simulink model "EV6_LUT_FourWheel_EV6Battery77p4kWh_PowerCorrected"  (R2024a)
settings: Solver=ode4  StartTime=0  StopTime=60  FixedStep=0.001  RelTol=1e-3
PreLoadFcn:
  | VSS_BICYCLE=Simulink.Variant('Dual=0');
  | VSS_DUAL=Simulink.Variant('Dual=1');
  | Dual=1;
  | load('DriveCycle2.mat')
PostLoadFcn:
  | if any(exist('dsrtsu_mdlpostloadfcn', 'file') ~= 0), dsrtsu_mdlpostloadfcn('Execute', bdroot); end
InitFcn:
  | , if any(exist('rtifpga_mdlclblib', 'file') ~= 0), rtifpga_mdlclblib('Init', bdroot); end,
  | , if any(exist('dsmpb_private', 'file') ~= 0), dsmpb_private('dsmpb_mdlclblib', 'Init', bdroot); end,
  | load('DriveCycle2.mat')
model workspace (MAT data in the model file):
  DiffRatio = 10.65
  EV6_2023_BattBranchCapacity_Ah = 55.5236728838
  EV6_2023_BattEnergy_kWh = 77.4
  EV6_2023_BattNominalVoltage_V = 697
  EV6_2023_BattNumCellsParallel = 2
  EV6_2023_BattNumCellsSeries = 192
  EV6_2023_BattOpenVoltCapBpts = [0 0.1 0.2 0.3 0.4 0.5 0.6 0.7 0.8 0.9 1]
  EV6_2023_BattOpenVoltTbl = [2.96762142548 3.40364281191 3.47417488548 3.54470541822 3.61523441014 3.68576186124 3.75628777151 3.82681214095 3.94527005036 4.07101207308 4.2120755254]
  EV6_2023_BattPackCapacity_Ah = 111.047345768
  EV6_2023_BattResistSocBpts = [0 0.2 0.4 0.6 0.8 1]
  EV6_2023_BattResistTbl = [0.0163620057716 0.0118174152018 0.00807187352333 0.00375663957972 0.00266904525531 0.00103635901355 0.0019014404175 0.0172368903217 0.0121226074867 0.00758541551769 0.00474065349228 0.00337561163613 ... (42 elements, 7x6)]
  EV6_2023_BattResistTempBpts = [243.1 253.1 263.1 273.1 283.1 298.1 313.1]
  EV6_2023_InitialPackOCV_V = 726.471714233
  EV6_2023_InitialSOC = 0.638878863672
  EV6_BattCellCapacity_Ah = 60.3
  EV6_BattInitialSOC = 0.638878863672
  EV6_BattOCV_Cell_V = [2.96762142548 3.40364281191 3.47417488548 3.54470541822 3.61523441014 3.68576186124 3.75628777151 3.82681214095 3.94527005036 4.07101207308 4.2120755254]
  EV6_BattOCV_SOC = [0 0.1 0.2 0.3 0.4 0.5 0.6 0.7 0.8 0.9 1]
  EV6_BattPackCapacity_Ah = 120.6
  EV6_BattParallelCells = 2
  EV6_BattResistanceSOC = [0 0.2 0.4 0.6 0.8 1]
  EV6_BattResistanceTable_Ohm = [0.0163620057716 0.0118174152018 0.00807187352333 0.00375663957972 0.00266904525531 0.00103635901355 0.0019014404175 0.0172368903217 0.0121226074867 0.00758541551769 0.00474065349228 0.00337561163613 ... (42 elements, 7x6)]
  EV6_BattResistanceTemp_K = [243.1 253.1 263.1 273.1 283.1 298.1 313.1]
  EV6_BattSeriesCells = 192
  EV6_FinalDriveRatio = 10.65
  EV6_TargetPackResistance_Ohm = 0.132763804608
  Gas = 0.383333333333
undefined symbols (not defined in the file): accel_bp_mps2, AccelCmd, ActTqLF_Nm_, ActTqLR_Nm_, ActTqRF_Nm_, ActTqRR_Nm_, BattChargeLimitMaxPwr, BattChargeLimitSocBpts, BattChargeLimitTbl, BattDischargeLimitSocBpts, BattDischargeLimitTbl, BattDischargeMaxPwr, BrakeMaxPrs, BrakeMaxTrq, ChassisDistCg2FrontAxle, ChassisDistCg2RearAxle, ChassisVehMass, CltchCmd, CoastDown, DecelCmd, DiscIntNeverNeededParam, EnvGravCnst, EnvPrs, EnvTemp, EV6_RegenTorqueGain, EV6_TractionTorqueGain, front_share_regen_3d, front_share_traction_3d, FuelSpecificGrav, GearCmd, h, InitStates, lgSw, limitedMCT, MCT, MtrEffSpdBpts, MtrEffTbl, MtrEffTrqBpts, MtrPwrMax, MtrTrqMax, out_1, pMCT, RealSimPara, Ref_speed, Ref_time, regen_torque_bp_Nm, speed_bp_kph, SteeringCmd, SupvsryCtrlRegenBrkCutOffTbl, SupvsryCtrlRegenSpdBpts, TestScnrioCycleNum, traction_torque_bp_Nm, US06, VEH
libraries: VSIGenLib x65, simulink x54, etargetslib x38, dsmpblib x24, vehdynlibtire x12, autolibshared x11, vehdynlibsuspension x7, vehdynlibtirecommon x7, autolibpowerinfoutils x6, autolibutils x5, autolibsharedcoupling x4, autolibmappedmotor x4
(part 5 of 19)

== system EV6_LUT_FourWheel_EV6Battery77p4kWh_PowerCorrected/Vehicle Under Test1/Vehicle/Motor_R ==
  SupvsryCtrl : Inport
  MtrSpd : Inport  Port=2
  Bus Creator1 : BusCreator  Inputs=1
  Bus Creator2 : BusCreator  Inputs=4
  Bus Selector1 : BusSelector  OutputSignals=Volt
  Bus Selector2 : BusSelector  OutputSignals=MtrTrqCmd
  Bus Selector3 : BusSelector  OutputSignals=PwrInfo.PwrTrnsfrd.PwrMtr,PwrInfo.PwrTrnsfrd.PwrBus
  Mach-E Motor : autolibmappedmotor/Mapped Motor  port_config=Speed  param_by=Maximum torque and power  w_t=[ 0 375 750 800 ]  T_t=[0.09 0.08 0.07 0]  torque_max=800  power_max=358000  Tc=0.01  param_loss=Tabulated efficiency data  eff=100  w_eff=375  T_eff=0.08  Piron=0  Pbase=0  w_eff_bp=MtrEffSpdBpts.*pi/30  T_eff_bp=MtrEffTrqBpts  Temp_eff_bp=[233.15 293.15 373.15]  losses_table=[1 2;3 4]  losses_table_3d=cat(3,[1.49 1.67 2.21 3.10; 0.42 0.69 1.14 2.03; 0.06 0.24 0.78 1.68; 0.42 0.69 1.14 2.03; 1.49 1.67 2.21 3.10],[1.49 1.67 2.21 3.10; 0.42 0.69 1.14 2.03; 0.06 0.24 0.78 1.68; 0.42 0.69 1.14 2.03; 1.49 1.67 2.21 3.10],[1.49 1.67 2.21 3.10; 0.42 0.69 1.14 2.03; 0.06 0.24 0.78 1.68; 0.42 0.69 1.14 2.03; 1.49 1.67 2.21 3.10])  efficiency_table=MtrEffTbl*0.94  efficiency_table_3d=cat(3,[95 95 95 95; 95 95 95 95; 95 95 95 95; 95 95 95 95; 95 95 95 95],[95 95 95 95; 95 95 95 95; 95 95 95 95; 95 95 95 95; 95 95 95 95],[95 95 95 95; 95 95 95 95; 95 95 95 95; 95 95 95 95; 95 95 95 95])  J=5e-6  b=1e-5  omega_o=0  T_t_extended=[0 0.07 0.08 0.09 0.08 0.07 0]  w_t_extended=[-800 -750 -375 0 375 750 800]  KLossIron=0  KLossCopper=0  x_w_eff_vec=[-1047.1975511966 -942.477796076938 -837.758040957278 -733.038285837618 -628.318530717959 -523.598775598299 -418.879020478639 -314.159265358979 -285.714285713875 -209.43951023932 -104.71975511966 0 104.71975511966 209.43951023932 285.714285713875 314.159265358979 418.879020478639 523.598775598299 628.318530717959 733.038285837618 837.758040957278 942.477796076938 1047.1975511966]  x_T_eff_vec=[-360 -334.285714285714 -308.571428571429 -282.857142857143 -257.142857142857 -231.428571428571 -205.714285714286 -180 -154.285714285714 -128.571428571429 -102.857142857143 -77.1428571428572 -51.4285714285714 -25.7142857142857 0 25.7142857142857 51.4285714285714 77.1428571428572 102.857142857143 128.571428571429 154.285714285714 180 205.714285714286 231.428571428571 257.142857142857 282.857142857143 308.571428571429 334.285714285714 360]  x_tmp_eff_vec=[-0.09 -0.06 -0.03 0 0.03 0.06 0.09]  x_losses_mat=[54250.1517943165 50375.1409518653 46500.1301094142 42625.119266963 38750.1084245118 34875.0975820605 31000.0867396095 27125.0758971582 23250.065054707 19375.054212256 15500.0433698047 12629.4764797412 9803.55154311708 6774.11181875432 0 5412.5153431847 8293.80460547705 10921.9712596802 13550.1379138833 16937.6723923542 20325.2068708249 23712.7413492957 27100.2758277666 30487.8103062373 33875.3447847082 37262.879263179 40650.4137416499 44037.9482201206 47425.4826985915;44696.230836134 41503.6429192672 38311.0550024006 35118.4670855338 31925.8791686671 28733.2912518003 25540.7033349337 22348.115418067 19155.5275012002 15962.9395843336 12770.3516674669 9577.76375060014 6975.01951641212 6096.70063687888 0 4871.26380886623 6097.56206124747 8462.91205003029 11283.8827333737 14104.8534167172 16925.8241000605 19746.794783404 22567.7654667475 25388.7361500908 28209.7068334343 31030.6775167777 33851.6482001212 36672.6188834645 39493.589566808;36137.1105685043 33555.8883850397 30974.6662015752 28393.4440181105 25812.2218346459 23230.9996511813 20649.7774677168 18068.5552842522 15487.3331007875 12906.110917323 10324.8887338584 8513.56777831124 6200.01734792188 5419.28945500345 0 4330.01227454776 5420.05516555331 7522.58848891581 9220.12563933554 11525.1570491694 13830.1884590033 16135.2198688372 18440.2512786711 20745.2826885049 23050.3140983388 25355.3455081727 27660.3769180066 29965.4083278404 32270.4397376744;31619.9717474413 29361.4023369097 27102.8329263783 24844.2635158467 22585.6941053152 20327.1246947836 18068.5552842522 15809.9858737206 13551.4164631891 11292.8470526576 9034.27764212609 7449.37180602233 5425.01517943165 4741.87827312802 0 3788.76074022929 4742.54826985915 6582.26492780134 8067.6099344186 10084.5124180233 12101.4149016279 14118.3173852325 16135.2198688372 18152.1223524418 20169.0248360465 22185.9273196511 24202.8298032558 26219.7322868604 28236.6347704651;27102.8329263782 25166.9162887798 23230.9996511814 21295.0830135829 19359.1663759844 17423.249738386 15487.3331007876 13551.4164631891 11615.4998255906 9679.58318799226 8513.56777831124 6385.17583373343 4650.01301094141 4064.46709125259 0 3247.50920591082 4065.04137416498 5641.94136668686 7522.58848891582 8643.86778687709 10372.6413442524 12101.4149016279 13830.1884590033 15558.9620163787 17287.7355737541 19016.5091311295 20745.282688505 22474.0562458803 24202.8298032558;22585.6941053152 20972.4302406498 19359.1663759845 17745.9025113191 16132.6386466537 14519.3747819883 12906.110917323 11292.8470526576 9679.58318799221 8066.31932332688 7094.63981525937 5320.97986144452 3875.01084245118 3387.05590937716 0 2706.25767159235 3387.53447847082 4701.61780557238 6268.82374076318 7203.22315573091 8643.86778687704 10084.5124180232 11525.1570491694 12965.8016803156 14406.4463114618 15847.0909426079 17287.7355737541 18728.3802049003 20169.0248360465;19864.9914827262 18446.0635196743 17027.1355566225 15608.2075935706 14189.2796305187 12770.3516674668 11351.423704415 9932.4957413631 8513.56777831121 7094.63981525938 5675.71185220749 4256.78388915562 3100.00867396094 2709.64472750173 0 2165.00613727388 2710.02758277665 3761.29424445791 5015.05899261055 6268.82374076319 7522.58848891579 8776.35323706844 10030.1179852211 11283.8827333737 12537.6474815263 13791.412229679 15045.1769778316 16298.9417259842 17552.7064741369;20587.4582405459 19116.9255090783 17646.3927776108 16175.8600461432 12629.4764797412 11366.528831767 10103.581183793 8137.52276914747 6975.01951641211 5812.51626367679 4650.01301094142 3788.84294392236 2525.89529594824 2032.23354562629 0 1623.75460295541 2184.39425193603 3276.59137790406 4065.04137416499 5081.30171770625 6097.56206124746 7113.82240478872 8737.57700774416 9829.77413371214 10921.9712596802 13684.7775990372 14928.8482898587 16172.9189806802 17416.9896715018;18723.4042552922 17386.0182370571 16048.6322188219 14711.2462005868 11485.9634880614 10337.3671392553 9188.77079044916 8040.174441643 6891.57809283685 5742.98174403074 4594.38539522458 ...(+6536 chars)]  x_losses_mat_3d=[37.8947368421052 25.2631578947368 12.6315789473684 0 12 24 36;18.9473684210526 12.6315789473684 6.3157894736842 0 5.99999999999999 12 18;0 0 0 0 0 0 0;18 12 5.99999999999999 0 6.3157894736842 12.6315789473684 18.9473684210526;36 24 12 0 12.6315789473684 25.2631578947368 37.8947368421052]  CalLossMapData={}  CalLossWithTempMapData={}  aMode=aMode  RefBlkName='autolibmappedmotor/Mapped Motor'
  Mapped Motor : autolibmappedmotor/Mapped Motor  port_config=Speed  param_by=Maximum torque and power  w_t=[ 0 375 750 800 ]  T_t=[0.09 0.08 0.07 0]  torque_max=MtrTrqMax  power_max=MtrPwrMax  Tc=MtrTrqTimeCnst  param_loss=Tabulated efficiency data  eff=100  w_eff=375  T_eff=0.08  Piron=0  Pbase=0  w_eff_bp=MtrEffSpdBpts.*pi/30  T_eff_bp=MtrEffTrqBpts  Temp_eff_bp=[233.15 293.15 373.15]  losses_table=[1 2;3 4]  losses_table_3d=cat(3,[1.49 1.67 2.21 3.10; 0.42 0.69 1.14 2.03; 0.06 0.24 0.78 1.68; 0.42 0.69 1.14 2.03; 1.49 1.67 2.21 3.10],[1.49 1.67 2.21 3.10; 0.42 0.69 1.14 2.03; 0.06 0.24 0.78 1.68; 0.42 0.69 1.14 2.03; 1.49 1.67 2.21 3.10],[1.49 1.67 2.21 3.10; 0.42 0.69 1.14 2.03; 0.06 0.24 0.78 1.68; 0.42 0.69 1.14 2.03; 1.49 1.67 2.21 3.10])  efficiency_table=MtrEffTbl*0.94  efficiency_table_3d=cat(3,[95 95 95 95; 95 95 95 95; 95 95 95 95; 95 95 95 95; 95 95 95 95],[95 95 95 95; 95 95 95 95; 95 95 95 95; 95 95 95 95; 95 95 95 95],[95 95 95 95; 95 95 95 95; 95 95 95 95; 95 95 95 95; 95 95 95 95])  J=5e-6  b=1e-5  omega_o=0  T_t_extended=[0 0.07 0.08 0.09 0.08 0.07 0]  w_t_extended=[-800 -750 -375 0 375 750 800]  KLossIron=0  KLossCopper=0  x_w_eff_vec=[-1047.1975511966 -942.477796076938 -837.758040957278 -733.038285837618 -628.318530717959 -523.598775598299 -418.879020478639 -314.159265358979 -285.714285713875 -209.43951023932 -104.71975511966 0 104.71975511966 209.43951023932 285.714285713875 314.159265358979 418.879020478639 523.598775598299 628.318530717959 733.038285837618 837.758040957278 942.477796076938 1047.1975511966]  x_T_eff_vec=[-360 -334.285714285714 -308.571428571429 -282.857142857143 -257.142857142857 -231.428571428571 -205.714285714286 -180 -154.285714285714 -128.571428571429 -102.857142857143 -77.1428571428572 -51.4285714285714 -25.7142857142857 0 25.7142857142857 51.4285714285714 77.1428571428572 102.857142857143 128.571428571429 154.285714285714 180 205.714285714286 231.428571428571 257.142857142857 282.857142857143 308.571428571429 334.285714285714 360]  x_tmp_eff_vec=[-0.09 -0.06 -0.03 0 0.03 0.06 0.09]  x_losses_mat=[54250.1517943165 50375.1409518653 46500.1301094142 42625.119266963 38750.1084245118 34875.0975820605 31000.0867396095 27125.0758971582 23250.065054707 19375.054212256 15500.0433698047 12629.4764797412 9803.55154311708 6774.11181875432 0 5412.5153431847 8293.80460547705 10921.9712596802 13550.1379138833 16937.6723923542 20325.2068708249 23712.7413492957 27100.2758277666 30487.8103062373 33875.3447847082 37262.879263179 40650.4137416499 44037.9482201206 47425.4826985915;44696.230836134 41503.6429192672 38311.0550024006 35118.4670855338 31925.8791686671 28733.2912518003 25540.7033349337 22348.115418067 19155.5275012002 15962.9395843336 12770.3516674669 9577.76375060014 6975.01951641212 6096.70063687888 0 4871.26380886623 6097.56206124747 8462.91205003029 11283.8827333737 14104.8534167172 16925.8241000605 19746.794783404 22567.7654667475 25388.7361500908 28209.7068334343 31030.6775167777 33851.6482001212 36672.6188834645 39493.589566808;36137.1105685043 33555.8883850397 30974.6662015752 28393.4440181105 25812.2218346459 23230.9996511813 20649.7774677168 18068.5552842522 15487.3331007875 12906.110917323 10324.8887338584 8513.56777831124 6200.01734792188 5419.28945500345 0 4330.01227454776 5420.05516555331 7522.58848891581 9220.12563933554 11525.1570491694 13830.1884590033 16135.2198688372 18440.2512786711 20745.2826885049 23050.3140983388 25355.3455081727 27660.3769180066 29965.4083278404 32270.4397376744;31619.9717474413 29361.4023369097 27102.8329263783 24844.2635158467 22585.6941053152 20327.1246947836 18068.5552842522 15809.9858737206 13551.4164631891 11292.8470526576 9034.27764212609 7449.37180602233 5425.01517943165 4741.87827312802 0 3788.76074022929 4742.54826985915 6582.26492780134 8067.6099344186 10084.5124180233 12101.4149016279 14118.3173852325 16135.2198688372 18152.1223524418 20169.0248360465 22185.9273196511 24202.8298032558 26219.7322868604 28236.6347704651;27102.8329263782 25166.9162887798 23230.9996511814 21295.0830135829 19359.1663759844 17423.249738386 15487.3331007876 13551.4164631891 11615.4998255906 9679.58318799226 8513.56777831124 6385.17583373343 4650.01301094141 4064.46709125259 0 3247.50920591082 4065.04137416498 5641.94136668686 7522.58848891582 8643.86778687709 10372.6413442524 12101.4149016279 13830.1884590033 15558.9620163787 17287.7355737541 19016.5091311295 20745.282688505 22474.0562458803 24202.8298032558;22585.6941053152 20972.4302406498 19359.1663759845 17745.9025113191 16132.6386466537 14519.3747819883 12906.110917323 11292.8470526576 9679.58318799221 8066.31932332688 7094.63981525937 5320.97986144452 3875.01084245118 3387.05590937716 0 2706.25767159235 3387.53447847082 4701.61780557238 6268.82374076318 7203.22315573091 8643.86778687704 10084.5124180232 11525.1570491694 12965.8016803156 14406.4463114618 15847.0909426079 17287.7355737541 18728.3802049003 20169.0248360465;19864.9914827262 18446.0635196743 17027.1355566225 15608.2075935706 14189.2796305187 12770.3516674668 11351.423704415 9932.4957413631 8513.56777831121 7094.63981525938 5675.71185220749 4256.78388915562 3100.00867396094 2709.64472750173 0 2165.00613727388 2710.02758277665 3761.29424445791 5015.05899261055 6268.82374076319 7522.58848891579 8776.35323706844 10030.1179852211 11283.8827333737 12537.6474815263 13791.412229679 15045.1769778316 16298.9417259842 17552.7064741369;20587.4582405459 19116.9255090783 17646.3927776108 16175.8600461432 12629.4764797412 11366.528831767 10103.581183793 8137.52276914747 6975.01951641211 5812.51626367679 4650.01301094142 3788.84294392236 2525.89529594824 2032.23354562629 0 1623.75460295541 2184.39425193603 3276.59137790406 4065.04137416499 5081.30171770625 6097.56206124746 7113.82240478872 8737.57700774416 9829.77413371214 10921.9712596802 13684.7775990372 14928.8482898587 16172.9189806802 17416.9896715018;18723.4042552922 17386.0182370571 16048.6322188219 14711.2462005868 11485.9634880614 10337.3671392553 9188.77079044916 8040.174441643 6891.57809283685 5742.98174403074 4594.38539522458 ...(+6536 chars)]  x_losses_mat_3d=[37.8947368421052 25.2631578947368 12.6315789473684 0 12 24 36;18.9473684210526 12.6315789473684 6.3157894736842 0 5.99999999999999 12 18;0 0 0 0 0 0 0;18 12 5.99999999999999 0 6.3157894736842 12.6315789473684 18.9473684210526;36 24 12 0 12.6315789473684 25.2631578947368 37.8947368421052]  CalLossMapData={}  CalLossWithTempMapData={}  aMode=aMode  RefBlkName='autolibmappedmotor/Mapped Motor'
  Memory : Memory
  Mux{,1..3} (4 alike) : Mux  Inputs=1
  Scope : Scope
  To Workspace : ToWorkspace  VariableName=MtrTrq_R_Mache  SaveFormat=Structure With Time  SampleTime=-1
  Two-Way Connection1 : TwoWayConnection
  Batt : PMIOPort  Side=Left
  Mtr : Outport
  MtrTrq : Outport  Port=2
  wires:
  MtrSpd/1 -> Mux1/1, Mach-E Motor/2
  Memory/1 -> Bus Creator1/1  "Curr"
  Mux3/1 -> Bus Creator2/4  "MtrElecPwr"
  Bus Selector3/2 -> Mux3/1  "<PwrBus>"
  Mux1/1 -> Bus Creator2/1  "MtrSpd"
  Bus Selector3/1 -> Mux2/1  "<PwrMtr>"
  Mux2/1 -> Bus Creator2/3  "MtrMechPwr"
  Bus Creator2/1 -> Mtr/1
  Mux/1 -> Bus Creator2/2  "MtrTrq"
  Bus Selector2/1 -> Scope/1, Mach-E Motor/3  "<MtrTrqCmd>"
  Bus Selector1/1 -> Mach-E Motor/1  "<Volt>"
  Two-Way Connection1/1 -> Bus Selector1/1
  SupvsryCtrl/1 -> Bus Selector2/1
  Mach-E Motor/1 -> Bus Selector3/1
  Bus Creator1/1 -> Two-Way Connection1/1
  Mach-E Motor/2 -> Memory/1  "Curr"
  Mach-E Motor/3 -> To Workspace/1, MtrTrq/1, Mux/1  "Trq"
  connections:
  Batt/RConn1 -- Two-Way Connection1/RConn1

== system EV6_LUT_FourWheel_EV6Battery77p4kWh_PowerCorrected/Vehicle Under Test1/Vehicle/Powertrain Supervisory Controller  ==
  Driver : Inport
  Chassis : Inport  Port=2
  Mtr : Inport  Port=3
  Batt : Inport  Port=4
  Accel Test Override : ManualSwitch
  Brake Test Override : ManualSwitch
  Bus Selector : BusSelector  OutputSignals=SteeringCmd
  Bus Selector1 : BusSelector  OutputSignals=ax
  Constant : Constant  Value=0
  Constant1 : Constant  Value=0.5
  Constant2 : Constant  Value=0.2
  Engine Torque Command : Subsystem
  Gain : Gain  Gain=9.80665
  Scope : Scope  NumInputPorts=4
  Step : Step  Time=5  Before=0.2  After=0  SampleTime=0
  Step1 : Step  Time=5  After=0.5  SampleTime=0
  Subsystem1 : Subsystem
      mask Display: disp('')
  Subsystem4 : Subsystem
      mask Display: disp('')
  Transfer Fcn : TransferFcn  Numerator=[12.566]  Denominator=[1 12.566]
  VehAcc : Display
  VehSpd entering ETC : Display
  SupvsryCtrl : Outport
  FrontMtrTrqCmd : Outport  Port=2
  RearMtrTrqCmd : Outport  Port=3
  wires:
  Bus Selector/1 -> Subsystem1/5(SteeringCmd)  "<SteeringCmd>"
  Driver/1 -> Subsystem4/1(Driver), Bus Selector/1
  Chassis/1 -> Bus Selector1/1, Subsystem4/2(Chassis)
  Batt/1 -> Subsystem4/3(Batt)
  Subsystem1/1(SupvsryCtrl) -> SupvsryCtrl/1
  Mtr/1 -> Subsystem4/4(Mtr)
  Subsystem4/3(DriverGearCmd) -> Engine Torque Command/3(DriverGearCmdIn)
  Subsystem4/4(VehSpd) -> VehSpd entering ETC/1, Engine Torque Command/4(VehSpd)
  Subsystem4/5(BattSoc) -> Engine Torque Command/5(BattSoc)
  Subsystem4/6(MtrSpd) -> Engine Torque Command/6(MtrSpd)
  Engine Torque Command/1(MtrTrqCmd) -> Scope/1, Subsystem1/1(MtrTrqCmd)  "MtrTrqCmd"
  Engine Torque Command/2(AccelCmd) -> Subsystem1/2(AccelCmd), Scope/2  "AccelCmd"
  Engine Torque Command/3(BrkCmd) -> Subsystem1/3(BrkCmd), Scope/3  "BrkCmd"
  Engine Torque Command/4(DriverGearCmd) -> Subsystem1/4(DriverGearCmd), Scope/4  "DriverGearCmd"
  Bus Selector1/1 -> VehAcc/1, Transfer Fcn/1  "<ax>"
  Transfer Fcn/1 -> Gain/1  "VehAcc_Filtered_g"
  Subsystem4/1(AccelCmd) -> Accel Test Override/1
  Accel Test Override/1 -> Engine Torque Command/1(AccelCmdIn)  "AccelCmd_ETC"
  Subsystem4/2(DecelCmd) -> Brake Test Override/1
  Brake Test Override/1 -> Engine Torque Command/2(DecelCmdIn)  "DecelCmd_ETC"
  Engine Torque Command/6(RearMtrTrqCmd) -> RearMtrTrqCmd/1
  Engine Torque Command/5(FrontMtrTrqCmd) -> FrontMtrTrqCmd/1
  Step/1 -> Accel Test Override/2
  Step1/1 -> Brake Test Override/2
  Gain/1 -> Engine Torque Command/7(VehAcc)  "VehAcc_LUT_Input_mps2"

== system EV6_LUT_FourWheel_EV6Battery77p4kWh_PowerCorrected/Vehicle Under Test1/Vehicle/Rear Wheel Drive ==
  DrvShfTrq : Inport
  Omega : Inport  Port=2
  Ideal Diff : Subsystem  VariantControl=0
  Ideal Diff AWD : Subsystem  VariantControl=Choice
  Real Diff : Subsystem  VariantControl=1
  Diff : Outport  VectorParamsAs1DForOutWhenUnconnected=off
  AxlTrq : Outport  Port=2  VectorParamsAs1DForOutWhenUnconnected=off
  PropShaftSpd : Outport  Port=3  VectorParamsAs1DForOutWhenUnconnected=off
  PropShaftSpd1 : Outport  Port=4

== system EV6_LUT_FourWheel_EV6Battery77p4kWh_PowerCorrected/Vehicle Under Test1/Vehicle/Rototest UDP RX ExternalMode   ==
  RotoTest ExternalControlEthernet : dsmpblib/Data Inport  Priority=10000
      settings: SourceProductName=dSPACE Model Interface Package for Simulink (MIPS)
  Terminator{1..5,10..11} (7 alike) : Terminator
  UDP Receive (1) : dsmpblib/Data Inport  Priority=10000
      settings: SourceProductName=dSPACE Model Interface Package for Simulink (MIPS)
  UDP Transmit (4)_In : dsmpblib/Data Inport  Priority=10000
      settings: SourceProductName=dSPACE Model Interface Package for Simulink (MIPS)
  Data Vector : Outport
  wires:
  RotoTest ExternalControlEthernet/1 -> Terminator1/1
  UDP Receive (1)/1 -> Data Vector/1
  UDP Transmit (4)_In/2 -> Terminator11/1
  UDP Receive (1)/2 -> Terminator2/1
  UDP Receive (1)/5 -> Terminator5/1
  UDP Transmit (4)_In/1 -> Terminator10/1
  UDP Receive (1)/3 -> Terminator3/1
  UDP Receive (1)/4 -> Terminator4/1

== system EV6_LUT_FourWheel_EV6Battery77p4kWh_PowerCorrected/Vehicle Under Test1/Vehicle/Rototest UDP TX ExternalMode   ==
  Rototest_UDP_TX : Inport
  UDP Transmit (4)_Out : dsmpblib/Data Outport  Priority=-10000
      settings: SourceProductName=dSPACE Model Interface Package for Simulink (MIPS)
  wires:
  Rototest_UDP_TX/1 -> UDP Transmit (4)_Out/1

== system EV6_LUT_FourWheel_EV6Battery77p4kWh_PowerCorrected/Vehicle Under Test1/Vehicle/Rototest and ORNL Interface ==
  note: rad/s
  CarTrqT2W : Inport
  UDP Input : Inport  Port=2
  BRAKE_PRESSED : Inport  Port=3
  vehSpeedKph : Inport  Port=4
  FXIN : Inport  Port=5
  1/tireRadius : Gain  Gain=1/0.3232
  ChargingMode : Constant  Value=0
  CmdSpeed (mph) : Constant  Value=0
  Constant : Constant  Value=3000
  DriverSwitch : Constant  Value=0
  DummyPT : Subsystem
  Format CM Powertrain Signals : Subsystem
  From Rototest : Subsystem
  Get Wheel Spd Cmd Based on Wheel Dynamics : Subsystem
  Multiport Switch : MultiPortSwitch  DataPortOrder=Zero-based contiguous  Inputs=2  zeroidx=on  SaturateOnIntegerOverflow=off  InputSameDT=off
  Multiport Switch1 : MultiPortSwitch  DataPortOrder=Zero-based contiguous  Inputs=2  zeroidx=on  SaturateOnIntegerOverflow=off  InputSameDT=off
  RotoTrqPreprocess : Subsystem
  Scope : Scope
  Scope1 : Scope
  Subsystem2 : Subsystem
  Terminator2 : Terminator
  To Rototest with Band-Aid : Subsystem
  mph2m/s : Gain  Gain=0.44704
  BrakeUpd : Outport
  Powertrain Out : Outport  Port=2
  DataSend : Outport  Port=3
  WhlSpd : Outport  Port=4
  wires:
  RotoTrqPreprocess/1(AxleTrqRoto) -> [AxlTrqRoto]
  vehSpeedKph/1 -> To Rototest with Band-Aid/4(Vehicle_Speed_kph)  "vehSpeedKph"
  From Rototest/2(AxlTrq) -> RotoTrqPreprocess/1(AxleTrqRaw), Subsystem2/1(AxlTorq)
  From Rototest/1(SpdAct) -> Terminator2/1
  UDP Input/1 -> From Rototest/1(Input)
  FXIN/1 -> Get Wheel Spd Cmd Based on Wheel Dynamics/5(FxIn)
  mph2m/s/1 -> 1/tireRadius/1
  1/tireRadius/1 -> Multiport Switch1/3
  CmdSpeed (mph)/1 -> mph2m/s/1
  ChargingMode/1 -> Multiport Switch1/1
  Multiport Switch1/1 -> Format CM Powertrain Signals/2(RotoWheelSpd)
  BRAKE_PRESSED/1 -> To Rototest with Band-Aid/3(BRAKE_PRESSED)
  Constant/1 -> [MaxRegen]
  To Rototest with Band-Aid/1(Out1) -> DataSend/1  "DataSend"
  DummyPT/1(WheelTorqueOut) -> Multiport Switch/3
  CarTrqT2W/1 -> Get Wheel Spd Cmd Based on Wheel Dynamics/2(Trq_T2W)
  Subsystem2/1(BrakeUpd) -> Format CM Powertrain Signals/1(BrakingTorques), Get Wheel Spd Cmd Based on Wheel Dynamics/1(BrakingTorques), BrakeUpd/1
  DriverSwitch/1 -> Multiport Switch/1
  Format CM Powertrain Signals/1(PowerTrainOutIdeal) -> Powertrain Out/1
  [AxlTrqRoto] -> To Rototest with Band-Aid/2(AxleTrq_roto_Nm)
  RotoTrqPreprocess/2(AxleTrqVeh) -> Multiport Switch/2, Format CM Powertrain Signals/3(AxlTrq)
  Multiport Switch/1 -> Get Wheel Spd Cmd Based on Wheel Dynamics/3(AxlTrq), Scope/1
  Get Wheel Spd Cmd Based on Wheel Dynamics/1(WhlSpdCmd) -> Multiport Switch1/2, DummyPT/1(WhlSpeedIn), Scope1/1, To Rototest with Band-Aid/1(SpeedCmd_rps), WhlSpd/1  "WhlSpdCmd"
  [MaxRegen] -> Format CM Powertrain Signals/4(MaxRegen)
  [MaxRegen] -> Get Wheel Spd Cmd Based on Wheel Dynamics/4(MaxRegen)

== system EV6_LUT_FourWheel_EV6Battery77p4kWh_PowerCorrected/Vehicle Under Test1/Vehicle/Vehicle Dynamics ==
  Env : Inport
  SupvsryCtrl : Inport  Port=2
  AxlTrq : Inport  Port=3
  Vehicle 14DOF : Subsystem  VariantControl=Veh14DOF
  Vehicle 7DOF : Subsystem  VariantControl=Veh7DOF
  Vehicle Longitudinal : Subsystem  VariantControl=VehLong
  Whl : Outport
  Chassis : Outport  Port=2
  RototestInput : Outport  Port=3

== system EV6_LUT_FourWheel_EV6Battery77p4kWh_PowerCorrected/RealSim1/ToRealSim/RealSim CreatBus/rgba2uint ==
  In1 : Inport
  Divide : Product  Inputs=**
  Sum of Elements : Sum  Inputs=+
  rgba bit operation : Constant  Value=[2^24,2^16,2^8,2^0]
  Out1 : Outport
  wires:
  Sum of Elements/1 -> Out1/1
  rgba bit operation/1 -> Divide/2
  In1/1 -> Divide/1
  Divide/1 -> Sum of Elements/1

== system EV6_LUT_FourWheel_EV6Battery77p4kWh_PowerCorrected/RealSim2/ToRealSim/RealSim CreatBus/rgba2uint ==
  In1 : Inport
  Divide : Product  Inputs=**
  Sum of Elements : Sum  Inputs=+
  rgba bit operation : Constant  Value=[2^24,2^16,2^8,2^0]
  Out1 : Outport
  wires:
  Sum of Elements/1 -> Out1/1
  rgba bit operation/1 -> Divide/2
  In1/1 -> Divide/1
  Divide/1 -> Sum of Elements/1

== system EV6_LUT_FourWheel_EV6Battery77p4kWh_PowerCorrected/Vehicle Under Test1/Environment/Ground Feedback/3D Engine ==
  Friction : Inport
  Ground Z Level : Inport  Port=2
  Bus Creator : BusCreator  Inputs=4
  Bus Creator2 : BusCreator  Inputs=4
  Bus Creator3 : BusCreator  Inputs=2
  Bus Selector : BusSelector  OutputSignals=HitLoc
  Data Type Conversion : DataTypeConversion  SaturateOnIntegerOverflow=off  RndMeth=Floor
  Demux : Demux
  Demux1 : Demux
  Passenger Vehicle Ray Trace Set : sim3dlib/Vehicle Terrain Sensor  Priority=1  ActorTag=SimulinkVehicle1  VehExtEn=Constant  TireRadiiExt=Constant  VehCntrLngthVal=0  TireRadiiVal=0  VehRayLngth=10  LfRayLngth=20  RfRayLngth=20  LrRayLngth=20  RrRayLngth=20  VehRayOffset=0  LfRayOffset=-1  RfRayOffset=-1  LrRayOffset=-1  RrRayOffset=-1  VehEn=on  LfEn=on  RfEn=on  LrEn=on  RrEn=on  DbgEn=off  Ts=.03  aMode=aMode
  Rate Transition : RateTransition
  Reshape10 : Reshape  OutputDimensionality=Row vector (2-D)
  Selector1 : Selector  InputPortWidth=5  IndexOptions=Index vector (dialog)  Indices=[2:5]  OutputSizes=1
  Signal Specification : SignalSpecification  Unit=m
  Signal Specification1 : SignalSpecification  Unit=1
  Terminator : Terminator
  Terminator1 : Terminator
  Terminator2 : Terminator
  Zend Select : Selector  NumberOfDimensions=2  InputPortWidth=3  IndexOptions=Select all,Index vector (dialog)  Indices=[1 3],3  OutputSizes=1,1
  Ground : Outport  VectorParamsAs1DForOutWhenUnconnected=off
  wires:
  Ground Z Level/1 -> Terminator/1
  Data Type Conversion/1 -> Signal Specification/1
  Friction/1 -> Signal Specification1/1
  Bus Creator3/1 -> Ground/1
  Bus Creator2/1 -> Bus Creator3/2  "mu"
  Demux1/2 -> Bus Creator2/2  "mu_FR"
  Demux1/4 -> Bus Creator2/4  "mu_RR"
  Demux1/3 -> Bus Creator2/3  "mu_RL"
  Bus Creator/1 -> Bus Creator3/1  "z"
  Demux1/1 -> Bus Creator2/1  "mu_FL"
  Signal Specification1/1 -> Demux1/1
  Signal Specification/1 -> Demux/1
  Demux/3 -> Bus Creator/3  "G_RL_z"
  Demux/4 -> Bus Creator/4  "G_RR_z"
  Demux/1 -> Bus Creator/1  "G_FL_z"
  Demux/2 -> Bus Creator/2  "G_FR_z"
  Rate Transition/1 -> Data Type Conversion/1
  Passenger Vehicle Ray Trace Set/1 -> Bus Selector/1
  Reshape10/1 -> Selector1/1
  Passenger Vehicle Ray Trace Set/3 -> Terminator2/1
  Passenger Vehicle Ray Trace Set/2 -> Terminator1/1
  Bus Selector/1 -> Zend Select/1  "<HitLoc>"
  Zend Select/1 -> Reshape10/1
  Selector1/1 -> Rate Transition/1

== system EV6_LUT_FourWheel_EV6Battery77p4kWh_PowerCorrected/Vehicle Under Test1/Environment/Ground Feedback/Constant ==
  Friction : Inport
  Ground Z Level : Inport  Port=2
  Bus Creator : BusCreator  Inputs=4
  Bus Creator2 : BusCreator  Inputs=4
  Bus Creator3 : BusCreator  Inputs=2
  Demux : Demux
  Demux1 : Demux
  Signal Specification : SignalSpecification  Unit=m
  Signal Specification1 : SignalSpecification  Unit=1
  Ground : Outport  VectorParamsAs1DForOutWhenUnconnected=off
  wires:
  Bus Creator3/1 -> Ground/1
  Signal Specification1/1 -> Demux1/1
  Friction/1 -> Signal Specification1/1
  Bus Creator2/1 -> Bus Creator3/2  "mu"
  Demux1/2 -> Bus Creator2/2  "mu_FR"
  Demux1/1 -> Bus Creator2/1  "mu_FL"
  Demux1/4 -> Bus Creator2/4  "mu_RR"
  Demux1/3 -> Bus Creator2/3  "mu_RL"
  Bus Creator/1 -> Bus Creator3/1  "z"
  Demux/2 -> Bus Creator/2  "G_FR_z"
  Demux/3 -> Bus Creator/3  "G_RL_z"
  Demux/1 -> Bus Creator/1  "G_FL_z"
  Demux/4 -> Bus Creator/4  "G_RR_z"
  Signal Specification/1 -> Demux/1
  Ground Z Level/1 -> Signal Specification/1

== system EV6_LUT_FourWheel_EV6Battery77p4kWh_PowerCorrected/Vehicle Under Test1/Vehicle/Actuation and Outputs/MOOG Brake Actuator ==
  Brake Pedal command [%] : Inport
  " CAN Settings" : Subsystem
  BrakePedal Target Position Manual Bypass : Constant  Value=0
  BrakePedal TargetPosition Bypass Enable : Constant  Value=0
  Bus Selector : BusSelector  OutputSignals=ControlWord,TargetPositionFinal_cnt
  Constant : Constant  Value=0
  Constant1 : Constant
  ControlWord bypass Enable : Constant  Value=0
  ControlWord bypass Override value : Constant  Value=0
  Data Type Conversion : DataTypeConversion  SaturateOnIntegerOverflow=off  RndMeth=Floor
  Data Type Conversion1 : DataTypeConversion  SaturateOnIntegerOverflow=off  RndMeth=Floor
  Data Type Conversion2 : DataTypeConversion  SaturateOnIntegerOverflow=off  RndMeth=Floor
  Data Type Conversion3 : DataTypeConversion  OutDataTypeStr=double  SaturateOnIntegerOverflow=off  RndMeth=Floor
  Discrete Transfer Fcn : DiscreteTransferFcn  Numerator=[0.0099502]  Denominator=[1 -0.9900498]
  Gain : Gain
  Gain1 : Gain
  Gain2 : Gain  Gain=10
  MOOG Interface : Subsystem
  RPDO3\ControlWord0\ISignal Value\ControlWord0 Value [BrakeAct_Config\Simulated ECUs\CANOpen_MOOG_02\Controller\TX\PDUs] : dsmpblib/Data Outport  Priority=-10000  Commented=on
      settings: SourceProductName=dSPACE Model Interface Package for Simulink (MIPS)
  RPDO3\ModesOfOperation\ISignal Value\ModesOfOperation Value [BrakeAct_Config\Simulated ECUs\CANOpen_MOOG_02\Controller\TX\PDUs] : dsmpblib/Data Outport  Priority=-10000  Commented=on
      settings: SourceProductName=dSPACE Model Interface Package for Simulink (MIPS)
  RPDO3\TargetPosition\ISignal Value\TargetPosition Value [BrakeAct_Config\Simulated ECUs\CANOpen_MOOG_02\Controller\TX\PDUs] : dsmpblib/Data Outport  Priority=-10000  Commented=on
      settings: SourceProductName=dSPACE Model Interface Package for Simulink (MIPS)
  Rate Limiter : RateLimiter  RisingSlewLimit=50  FallingSlewLimit=-50  SampleTimeMode=inherited
  Sine Wave : Sin  Amplitude=50  Bias=50  SampleTime=0
  Switch : Switch  Criteria=u2 > Threshold  SaturateOnIntegerOverflow=off  InputSameDT=off
  Switch1 : Switch  Criteria=u2 > Threshold  SaturateOnIntegerOverflow=off  InputSameDT=off
  Switch2 : Switch  Criteria=u2 > Threshold  SaturateOnIntegerOverflow=off  InputSameDT=off
  TPDO3\ActualPosition\ISignal Value\ActualPosition Value [BrakeAct_Config\Simulated ECUs\CANOpen_MOOG_02\Controller\RX\PDUs] : dsmpblib/Data Inport  Priority=10000  Commented=on
      settings: SourceProductName=dSPACE Model Interface Package for Simulink (MIPS)
  TPDO3\ModesOfOperationDisplay\ISignal Value\ModesOfOperationDisplay Value [BrakeAct_Config\Simulated ECUs\CANOpen_MOOG_02\Controller\RX\PDUs] : dsmpblib/Data Inport  Priority=10000  Commented=on
      settings: SourceProductName=dSPACE Model Interface Package for Simulink (MIPS)
  TPDO3\StatusWord0\ISignal Value\StatusWord0 Value [BrakeAct_Config\Simulated ECUs\CANOpen_MOOG_02\Controller\RX\PDUs] : dsmpblib/Data Inport  Priority=10000  Commented=on
      settings: SourceProductName=dSPACE Model Interface Package for Simulink (MIPS)
  Terminator{,1..5} (6 alike) : Terminator
  constant : Constant
  trace selection : Constant  Value=0
  wires:
  Data Type Conversion/1 -> Terminator3/1
  Switch2/1 -> Gain/1
  Rate Limiter/1 -> Switch/3
  Gain1/1 -> Gain2/1, Terminator2/1  "BrakePedal_CmdFinal_pct"
  " CAN Settings"/1(CAN_CommsOK_Flg) -> MOOG Interface/1(CAN_CommsOK_Flg)
  Brake Pedal command [%]/1 -> Switch2/3
  ControlWord bypass Enable/1 -> Switch1/2
  BrakePedal Target Position Manual Bypass/1 -> Rate Limiter/1
  ControlWord bypass Override value/1 -> Switch1/1
  Bus Selector/1 -> Switch1/3  "<ControlWord>"
  Switch1/1 -> Data Type Conversion1/1
  Gain/1 -> MOOG Interface/2(TargetPosition [pct])  "BrakePedal_TargetlPosition_pct"
  Data Type Conversion1/1 -> Terminator4/1  "ControlWord_Final"
  trace selection/1 -> Switch/2
  BrakePedal TargetPosition Bypass Enable/1 -> Switch2/2
  constant/1 -> Data Type Conversion/1
  Data Type Conversion2/1 -> Terminator5/1, Gain1/1  "TargetPosition_Cnt_Final"
  Sine Wave/1 -> Switch/1
  MOOG Interface/3(BrakeActuatorReady) -> Terminator1/1  "BrakeActuator_Ready_bool"
  Bus Selector/2 -> Data Type Conversion2/1  "<TargetPositionFinal_cnt>"
  MOOG Interface/2(ActualPosition [pct]) -> Terminator/1  "BrakePedal_ActualPosition_pct"
  MOOG Interface/1(Commands) -> Bus Selector/1
  Switch/1 -> Switch2/1
  Constant/1 -> MOOG Interface/3(StatusWord in)
  Constant1/1 -> MOOG Interface/5(Mode of operation in)
  Gain2/1 -> Data Type Conversion3/1
  Data Type Conversion3/1 -> Discrete Transfer Fcn/1
  Discrete Transfer Fcn/1 -> MOOG Interface/4(ActualPosition_cnt in)

== system EV6_LUT_FourWheel_EV6Battery77p4kWh_PowerCorrected/Vehicle Under Test1/Vehicle/Actuation and Outputs/Vehicle Accel Pedal Voltage Output ==
  APP_pct : Inport
  APP1Tbl : Lookup_n-D  NumberOfTableDimensions=1  BreakpointsForDimension1=[0 100]  Table=[16 78.8]  InternalRulePriority=Speed  RndMeth=Simplest
  APP2Tbl : Lookup_n-D  NumberOfTableDimensions=1  BreakpointsForDimension1=[0 100]  Table=[8 39.4]  InternalRulePriority=Speed  RndMeth=Simplest
  AccelPosition Bypass Enable : Constant  Value=0
  AccelPosition Manual Bypass [%] : Constant  Value=0
  Gain : Gain
  Gain1 : Gain
  Gain2 : Gain
  Gain3 : Gain  Gain=1/100
  Gain4 : Gain  Gain=1/100
  Product2 : Product
  Product3 : Product
  Rate Limiter : RateLimiter  RisingSlewLimit=50  FallingSlewLimit=-50  SampleTimeMode=inherited
  Switch2 : Switch  Criteria=u2 > Threshold  SaturateOnIntegerOverflow=off  InputSameDT=off
  Terminator2 : Terminator
  VRef : Constant  Value=5.01
  Voltage Out (1) : dsmpblib/Data Outport  Priority=-10000  Commented=on
      settings: SourceProductName=dSPACE Model Interface Package for Simulink (MIPS)
  Voltage Out (2) : dsmpblib/Data Outport  Priority=-10000  Commented=on
      settings: SourceProductName=dSPACE Model Interface Package for Simulink (MIPS)
  APP1_CmdFinal_V : Outport
  APP2_CmdFinal_V1 : Outport  Port=2
  wires:
  APP1Tbl/1 -> Gain3/1
  Product3/1 -> Gain/1
  Gain3/1 -> Product2/1
  APP2Tbl/1 -> Gain4/1
  Product2/1 -> Gain1/1
  Gain4/1 -> Product3/2
  VRef/1 -> Product3/1, Product2/2
  Rate Limiter/1 -> Switch2/1
  Gain2/1 -> Terminator2/1  "AccelPedal_CmdFinal_pct"
  Gain1/1 -> APP1_CmdFinal_V/1  "APP1_CmdFinal_V"
  Gain/1 -> APP2_CmdFinal_V1/1  "APP2_CmdFinal_V"
  AccelPosition Bypass Enable/1 -> Switch2/2
  AccelPosition Manual Bypass [%]/1 -> Rate Limiter/1
  APP_pct/1 -> Switch2/3
  Switch2/1 -> Gain2/1, APP2Tbl/1, APP1Tbl/1  "APP_CmdFinal_pct"
